simulink model "simulink_flightgear_control_trim_wind_5"  (R2023a)
settings: Solver=VariableStepAuto  StartTime=0  StopTime=inf  FixedStep=0.1  RelTol=1e-3
values from neighbouring files (symbols this model uses):
  alpha = -5:0.1:25    [Boeing747model.m]
  alpha1 = 0:0.1:14    [Boeing747model.m]
  alpha2 = -5:0.1:25    [Boeing747model.m]
  alpha3 = -5:0.1:17    [Boeing747model.m]
  beta = -15:0.1:15    [Boeing747model.m]
  CL = 0:0.01:1.4    [Boeing747model.m]
  da = 0:1:20    [Boeing747model.m]
  dr = [0 5 10 15 20 25]    [Boeing747model.m]
  EPR_ = 0:0.1:1.8    [Boeing747model.m]    (also in engine.m)
  flap = [0 10 20 25 30]    [Boeing747model.m]
  high1 = 0:10000:40000    [Boeing747model.m]
  high2 = 0:20000:40000    [Boeing747model.m]
  high3 = [0 15000 25000 35000 40000]    [Boeing747model.m]    (also in engine.m)
  high4 = [0 10000 20000 40000]    [Boeing747model.m]
  interp_result = table2array(resultTable(:,2:end))    [Boeing747model.m]
  interp_result_mach = 0:0.1:0.9    [Boeing747model.m]
  interp_result_N1 = 80:5:110    [Boeing747model.m]
  m2ft = 3.280839895013    (= 3.28083989501)    [Boeing747model.m]    (also in engine.m)
  mach = 0:0.02:0.9    [Boeing747model.m]    (also in engine.m)
  mach1 = [0 0.3 0.5 0.7 0.8 0.84 0.86 0.88 0.9]    [Boeing747model.m]
  mach2 = [0 0.3 0.5 0.7 0.8 0.9]    [Boeing747model.m]
  mach3 = [0 0.1 0.3 0.5 0.6 0.7 0.8 0.9]    [Boeing747model.m]    (also in engine.m = [0 0.1 0.3 0.5  0.7 0.8 0.9])
  mach5 = [0 0.6 0.8 0.85 0.9]    [Boeing747model.m]
  mach6 = [0 0.6 0.8 0.9]    [Boeing747model.m]
  mach7 = [0 0.3 0.5 0.74 0.8 0.84 0.86 0.88 0.9]    [Boeing747model.m]
  mach8 = [0 0.3 0.5 0.74 0.8 0.84 0.86 0.88 0.9]    [Boeing747model.m]
  model = 'simulink_flightgear_control_trim_wind_5'    [traimcode.m]
  ms2kts = 1.943844492609    (= 1.94384449261)    [Boeing747model.m]    (also in engine.m)
  powerangle_ = 0:1:130    [Boeing747model.m]    (also in engine.m)
  T = [-45 0 60 120]    [Boeing747model.m]    (also in engine.m)
  V_E = 0:20:250    [Boeing747model.m]
undefined symbols (not defined in the file or in its folder): Earth, F, ft, Light, m, MIL, Model, Newton, P3DAERO, Raphson, Receive, s, Send, Unit, WGS84, Wind
libraries: simulink_extras x115, aerolibconvert2 x16, simulink x4, aerolibfltsims x3, shared6dof x1, aerolibasang x1, aerolibtransform2 x1, aerolibatmos2 x1, aerolibobsolete x1, aerolibwind2 x1
(part 5 of 5)

== system simulink_flightgear_control_trim_wind_5/Plane/气动系数/Subsystem58/Subsystem68 ==
  In1 : Inport
  In2 : Inport  Port=2
  Radians in : Inport  Port=3
  In4 : Inport  Port=4
  In5 : Inport  Port=5
  In6 : Inport  Port=6
  1-D Lookup Table54 : Lookup_n-D  NumberOfTableDimensions=1  BreakpointsForDimension1=P3DAERO.Cl_ai_mach(1,:)  Table=P3DAERO.Cl_ai_mach(2,:)  InternalRulePriority=Speed  RndMeth=Simplest
  2-D Lookup Table10 : Lookup_n-D  BreakpointsForDimension1=flap  BreakpointsForDimension2=alpha  Table=P3DAERO.delta_Cl_ai  InternalRulePriority=Speed  RndMeth=Simplest
      settings: InputPortMap=u0,u1
  2-D Lookup Table11 : Lookup_n-D  BreakpointsForDimension1=high1  BreakpointsForDimension2=mach  Table=P3DAERO.Cl_ai_aeroelastic  InternalRulePriority=Speed  RndMeth=Simplest
      settings: InputPortMap=u0,u1
  2-D Lookup Table9 : Lookup_n-D  BreakpointsForDimension1=flap  BreakpointsForDimension2=da  Table=P3DAERO.k_delta_ai  InternalRulePriority=Speed  RndMeth=Simplest
      settings: InputPortMap=u0,u1
  Abs : Abs  SaturateOnIntegerOverflow=off
  Constant16 : Constant  Value=-1
  Constant18 : Constant
  Constant20 : Constant  Value=2
  Gain3 : Gain  Gain=m2ft
  Product4 : Product  Inputs=3
  Product5 : Product  Inputs=5
  Radians to Degrees26 : simulink_extras/Transformations/Radians to Degrees
  Radians to Degrees9 : simulink_extras/Transformations/Radians to Degrees
  Saturation8 : Saturate  UpperLimit=20  LowerLimit=0
  Scope1 : Scope
  Scope4 : Scope
  Switch2 : Switch  SaturateOnIntegerOverflow=off  InputSameDT=off
  Out1 : Outport
  wires:
  In5/1 -> Switch2/2, Abs/1
  1-D Lookup Table54/1 -> Product5/1
  Switch2/1 -> Product4/3
  2-D Lookup Table10/1 -> Product5/2
  2-D Lookup Table11/1 -> Product5/3
  2-D Lookup Table9/1 -> Product5/4
  Radians to Degrees26/1 -> Saturation8/1
  In1/1 -> 2-D Lookup Table11/2, 1-D Lookup Table54/1
  In6/1 -> Product5/5
  Gain3/1 -> 2-D Lookup Table11/1
  Product5/1 -> Scope4/1, Product4/2
  Radians to Degrees9/1 -> 2-D Lookup Table10/2
  Constant16/1 -> Switch2/1
  In2/1 -> 2-D Lookup Table9/1, 2-D Lookup Table10/1
  Saturation8/1 -> 2-D Lookup Table9/2
  Constant20/1 -> Product4/1
  Constant18/1 -> Switch2/3
  Radians in/1 -> Radians to Degrees9/1
  In4/1 -> Gain3/1
  Product4/1 -> Scope1/1, Out1/1
  Abs/1 -> Radians to Degrees26/1

== system simulink_flightgear_control_trim_wind_5/Plane/气动系数/Subsystem58/Subsystem69 ==
  In1 : Inport
  Radians in : Inport  Port=2
  Gain : Gain  Gain=-0.0003
  Product15 : Product
  Radians to Degrees2 : simulink_extras/Transformations/Radians to Degrees
  Scope47 : Scope
  Out1 : Outport
  wires:
  Gain/1 -> Product15/2
  Radians to Degrees2/1 -> Gain/1
  Product15/1 -> Out1/1, Scope47/1
  Radians in/1 -> Radians to Degrees2/1
  In1/1 -> Product15/1

== system simulink_flightgear_control_trim_wind_5/Plane/气动系数/Subsystem58/Subsystem7 ==
  note: 低速模式
  note: 高速模式
  In1 : Inport
  In2 : Inport  Port=2
  In3 : Inport  Port=3
  In4 : Inport  Port=4
  In5 : Inport  Port=5
  2-D Lookup Table6 : Lookup_n-D  BreakpointsForDimension1=flap  BreakpointsForDimension2=V_E  Table=P3DAERO.dot_CL_dot_nz_lowspeed  InternalRulePriority=Speed  RndMeth=Simplest
      settings: InputPortMap=u0,u1
  2-D Lookup Table7 : Lookup_n-D  BreakpointsForDimension1=high1  BreakpointsForDimension2=mach  Table=P3DAERO.dot_CL_dot_nz_highspeed  InternalRulePriority=Speed  RndMeth=Simplest
      settings: InputPortMap=u0,u1
  Product4 : Product
  Scope7 : Scope
  Velocity Conversion : aerolibconvert2/Velocity Conversion  IU=m/s  OU=ft/s
  Out1 : Outport
  wires:
  In5/1 -> 2-D Lookup Table7/2
  Product4/1 -> Out1/1, Scope7/1
  In2/1 -> 2-D Lookup Table6/1
  In3/1 -> 2-D Lookup Table6/2
  2-D Lookup Table7/1 -> Product4/2
  In1/1 -> Product4/1
  In4/1 -> Velocity Conversion/1
  Velocity Conversion/1 -> 2-D Lookup Table7/1

== system simulink_flightgear_control_trim_wind_5/Plane/气动系数/Subsystem58/Subsystem8 ==
  note: 米变英尺
  note: 襟翼角度
  In1 : Inport
  In2 : Inport  Port=2
  Radians in : Inport  Port=3
  1-D Lookup Table97 : Lookup_n-D  NumberOfTableDimensions=1  BreakpointsForDimension1=P3DAERO.k_ge(1,:)  Table=P3DAERO.k_ge(2,:)  InternalRulePriority=Speed  RndMeth=Simplest
  2-D Lookup Table18 : Lookup_n-D  BreakpointsForDimension1=flap  BreakpointsForDimension2=alpha1  Table=P3DAERO.delta_CL_ge  InternalRulePriority=Speed  RndMeth=Simplest
      settings: InputPortMap=u0,u1
  Constant24 : Constant  Value=0
  Product16 : Product
  Radians to Degrees10 : simulink_extras/Transformations/Radians to Degrees
  Saturation3 : Saturate  UpperLimit=14  LowerLimit=0
  Scope48 : Scope
  Scope49 : Scope
  Switch12 : Switch  Criteria=u2 > Threshold  Threshold=24  SaturateOnIntegerOverflow=off  InputSameDT=off
  Velocity Conversion : aerolibconvert2/Velocity Conversion  IU=m/s  OU=ft/s
  Out1 : Outport
  wires:
  Radians to Degrees10/1 -> Saturation3/1
  Product16/1 -> Switch12/3
  Velocity Conversion/1 -> 1-D Lookup Table97/1
  Constant24/1 -> Switch12/1
  Saturation3/1 -> 2-D Lookup Table18/2
  Switch12/1 -> Out1/1, Scope49/1
  2-D Lookup Table18/1 -> Product16/2
  1-D Lookup Table97/1 -> Product16/1, Scope48/1
  Radians in/1 -> Radians to Degrees10/1
  In2/1 -> 2-D Lookup Table18/1
  In1/1 -> Velocity Conversion/1, Switch12/2

== system simulink_flightgear_control_trim_wind_5/Plane/气动系数/Subsystem58/Subsystem9 ==
  note: 地效修正
  note: 米变英尺
  note: 襟翼角度
  In1 : Inport
  In2 : Inport  Port=2
  Radians in : Inport  Port=3
  1-D Lookup Table59 : Lookup_n-D  NumberOfTableDimensions=1  BreakpointsForDimension1=P3DAERO.k_ge(1,:)  Table=P3DAERO.k_ge(2,:)  InternalRulePriority=Speed  RndMeth=Simplest
  2-D Lookup Table12 : Lookup_n-D  BreakpointsForDimension1=flap  BreakpointsForDimension2=alpha1  Table=P3DAERO.F_rho_ge  InternalRulePriority=Speed  RndMeth=Simplest
      settings: InputPortMap=u0,u1
  Constant18 : Constant
  Product12 : Product
  Radians to Degrees6 : simulink_extras/Transformations/Radians to Degrees
  Saturation1 : Saturate  UpperLimit=14  LowerLimit=0
  Scope31 : Scope
  Scope33 : Scope
  Sum11 : Sum
  Switch4 : Switch  Criteria=u2 > Threshold  Threshold=24  SaturateOnIntegerOverflow=off  InputSameDT=off
  Velocity Conversion : aerolibconvert2/Velocity Conversion  IU=m/s  OU=ft/s
  Out1 : Outport
  Out2 : Outport  Port=2
  wires:
  In2/1 -> 2-D Lookup Table12/1
  Radians to Degrees6/1 -> Saturation1/1
  Switch4/1 -> Out1/1, Scope31/1
  Velocity Conversion/1 -> 1-D Lookup Table59/1
  Saturation1/1 -> 2-D Lookup Table12/2
  Sum11/1 -> Switch4/3
  Constant18/1 -> Sum11/1, Switch4/1
  2-D Lookup Table12/1 -> Product12/1
  1-D Lookup Table59/1 -> Product12/2, Out2/1, Scope33/1
  Product12/1 -> Sum11/2
  Radians in/1 -> Radians to Degrees6/1
  In1/1 -> Velocity Conversion/1, Switch4/2

== matlab function simulink_flightgear_control_trim_wind_5/Plane/发动机/MATLAB Function2 ==
  data: flap input; site output; ma input
function site= fcn(flap,ma)
if(ma>=0&&ma<=0.25)
    if(flap==0)
    site=0;
    elseif (flap>0.1&&flap<=0.25)
        site=1;
    elseif(flap>0.25&&flap<=0.5)
        site=2;
    elseif(flap>0.5&&flap<=0.75)
        site=3;
    elseif(flap>0.75&&flap<=1)
        site=4;
    else
    site=0;
    end
elseif(ma>0.25&&ma<=0.35)
    if(flap==0)
    site=0;
    elseif(flap>0.1&&flap<=0.25)
        site=1;
    elseif(flap>0.25&&flap<=0.5)
        site=2;
    elseif(flap>0.5)
        site=3;
    else
    site=0;
    end
else
    site=0;
end

== matlab function simulink_flightgear_control_trim_wind_5/Plane/重量//惯量/MATLAB Function1 ==
  data: ixx input; y output; iyy input; izz input; ixz input
function y = fcn(ixx,iyy,izz,ixz)
I=[ixx  0  -ixz;
    0  iyy  0;
    -ixz 0   izz];
y = I;

== matlab function simulink_flightgear_control_trim_wind_5/Plane/MATLAB Function ==
  data: u input; y output
function y = fcn(u)

y = [(25-u)/100*8.32,0,0]';

== matlab function simulink_flightgear_control_trim_wind_5/Plane/气动系数/MATLAB Function ==
  data: u input; y output
function y = fcn(u)

x = [cosd(u) 0 -sind(u); %x为稳定轴系到体轴系的转换
    0       1      0 ;
    sind(u) 0  cosd(u)];

y=x';                  %y为体轴系到稳定轴系的转换

== matlab function simulink_flightgear_control_trim_wind_5/Plane/大气环境/气压高度+摄氏度偏差版本1 ==
  data: T output; p output; rho output; Hp input; a output; delta_ISA input; delta output; theta output; sigma output; Hd_m output; Hd_ft output
% File: isa_atmosphere_pressure_altitude_delta.m
%
% 输入:
%   Hp        气压高度 / pressure altitude (m) [0–84.852 km]
%   delta_ISA 温度偏差 (degC)，比如 -40 表示 ISA -40
%
% 输出:
%   T     实际温度 (K)，即 T_ISA(Hp) + delta_ISA
%   p     静压 (Pa)，由气压高度按 ISA 标准大气确定
%   rho   实际密度 (kg/m^3)，由 p 和 T 计算
%   a     实际声速 (m/s)，由 T 计算
%   delta 压力比 p/p0
%   theta 温度比 T/T0
%   sigma 密度比 rho/rho0
%   Hd_m  密度高度 (m)
%   Hd_ft 密度高度 (ft)

function [T, p, rho, a, delta, theta, sigma, Hd_m, Hd_ft] = isa_atmosphere_pressure_altitude_delta(Hp, delta_ISA)

    % 常数
    g0 = 9.80665;        % m/s^2
    R  = 287.05287;      % J/(kg*K)
    gamma = 1.4;         % 空气比热比

    p0 = 101325;         % Pa
    T0 = 288.15;         % K
    rho0 = 1.225;        % kg/m^3

    % ISA 分层参数
    h_base = [0, 11000, 20000, 32000, 47000, 51000, 71000, 84852]; % m
    L      = [-0.0065, 0.0, 0.0010, 0.0028, 0.0, -0.0028, -0.0020]; % K/m

    % 输入检查
    if any(Hp(:) < 0) || any(Hp(:) > 84852)
        error('Hp must be within [0, 84852] m.');
    end

    if isscalar(delta_ISA)
        delta_ISA = delta_ISA .* ones(size(Hp));
    elseif ~isequal(size(delta_ISA), size(Hp))
        error('delta_ISA must be scalar or the same size as Hp.');
    end

    T_ISA = zeros(size(Hp));
    p     = zeros(size(Hp));

    % 对每一个气压高度计算 ISA 温度和 ISA 压力
    for i = 1:numel(Hp)

        h = Hp(i);

        T_curr = T0;
        p_curr = p0;

        for j = 1:length(L)

            h1 = h_base(j);
            h2 = h_base(j+1);

            if h <= h2

                if L(j) == 0
                    T_layer = T_curr;
                    p(i) = p_curr * exp(-g0 * (h - h1) / (R * T_layer));
                else
                    T_layer = T_curr + L(j) * (h - h1);
                    p(i) = p_curr * (T_layer / T_curr)^(-g0 / (R * L(j)));
                end

                T_ISA(i) = T_layer;
                break;

            else

                if L(j) == 0
                    T_next = T_curr;
                    p_curr = p_curr * exp(-g0 * (h2 - h1) / (R * T_curr));
                else
                    T_next = T_curr + L(j) * (h2 - h1);
                    p_curr = p_curr * (T_next / T_curr)^(-g0 / (R * L(j)));
                end

                T_curr = T_next;
            end
        end
    end

    % 实际温度：ISA 温度 + ΔISA
    T = T_ISA + delta_ISA;

    if any(T(:) <= 0)
        error('Computed temperature is non-physical. T must be greater than 0 K.');
    end

    % 实际密度和声速
    rho = p ./ (R .* T);
    a   = sqrt(gamma * R .* T);

    % 无量纲比值
    delta = p ./ p0;
    theta = T ./ T0;
    sigma = rho ./ rho0;

    % 密度高度
    Hd_m = density_altitude_from_rho(rho);
    Hd_ft = Hd_m * 3.280839895;
end


function Hd = density_altitude_from_rho(rho_target)

    h_low  = -3048;   % -10000 ft
    h_high = 15240;   %  50000 ft

    Hd = zeros(size(rho_target));

    for i = 1:numel(rho_target)
        lo = h_low;
        hi = h_high;

        for k = 1:60
            mid = 0.5 * (lo + hi);
            rho_mid = isa_density(mid);

            if rho_mid > rho_target(i)
                lo = mid;
            else
                hi = mid;
            end
        end

        Hd(i) = 0.5 * (lo + hi);
    end
end


function rho = isa_density(h)
    [T, p] = isa_standard_Tp(h);
    R = 287.05287;
    rho = p / (R * T);
end


function [T, p] = isa_standard_Tp(h)

    g0 = 9.80665;
    R  = 287.05287;

    p0 = 101325;
    T0 = 288.15;

    h_base = [0, 11000, 20000, 32000, 47000, 51000, 71000, 84852];
    L      = [-0.0065, 0.0, 0.0010, 0.0028, 0.0, -0.0028, -0.0020];

    % 默认赋值，避免 Simulink Coder 认为输出未赋值
    T = T0;
    p = p0;

    T_curr = T0;
    p_curr = p0;

    for j = 1:length(L)
        h1 = h_base(j);
        h2 = h_base(j+1);

        if h <= h2
            if L(j) == 0
                T = T_curr;
                p = p_curr * exp(-g0 * (h - h1) / (R * T));
            else
                T = T_curr + L(j) * (h - h1);
                p = p_curr * (T / T_curr)^(-g0 / (R * L(j)));
            end
            return;
        else
            if L(j) == 0
                T_next = T_curr;
                p_curr = p_curr * exp(-g0 * (h2 - h1) / (R * T_curr));
            else
                T_next = T_curr + L(j) * (h2 - h1);
                p_curr = p_curr * (T_next / T_curr)^(-g0 / (R * L(j)));
            end

            T_curr = T_next;
        end
    end

    % 兜底路径，给 Coder 明确输出
    T = T_curr;
    p = p_curr;
end

== matlab function simulink_flightgear_control_trim_wind_5/Plane/气动系数/Subsystem58/Subsystem32/MATLAB Function15 ==
  data: u input; y output
function y = fcn(u)
%计算kq
y=-0.012*(u-25)+1;

== matlab function simulink_flightgear_control_trim_wind_5/Plane/大气环境/气压高度+摄氏度偏差版本 ==
  data: T output; p output; rho output; Hp input; a output; delta_ISA input; delta output; theta output; sigma output
% File: isa_atmosphere_pressure_altitude_delta.m
%
% 输入:
%   Hp        气压高度 / pressure altitude (m) [0–84.852 km]
%   delta_ISA 温度偏差 (°C)，比如 -40 表示 ISA -40
%
% 输出:
%   T     实际温度 (K)，即 T_ISA(Hp) + delta_ISA
%   p     静压 (Pa)，由气压高度按 ISA 标准大气确定
%   rho   实际密度 (kg/m^3)，由 p 和 T 计算
%   a     实际声速 (m/s)，由 T 计算
%
% 可选输出:
%   delta 压力比 p/p0
%   theta 温度比 T/T0
%   sigma 密度比 rho/rho0

function [T, p, rho, a, delta, theta, sigma] = isa_atmosphere_pressure_altitude_delta(Hp, delta_ISA)

    % 常数
    g0 = 9.80665;        % m/s^2
    R  = 287.05287;      % J/(kg·K)
    gamma = 1.4;         % 空气比热比

    p0 = 101325;         % Pa
    T0 = 288.15;         % K
    rho0 = 1.225;        % kg/m^3

    % ISA 分层参数
    % 注意：这里 Hp 按标准大气的高度层处理
    h_base = [0, 11000, 20000, 32000, 47000, 51000, 71000, 84852]; % m
    L      = [-0.0065, 0.0, 0.0010, 0.0028, 0.0, -0.0028, -0.0020]; % K/m

    % 输入检查
    if any(Hp(:) < 0) || any(Hp(:) > 84852)
        error('Hp must be within [0, 84852] m.');
    end

    % 允许 delta_ISA 为标量或与 Hp 同尺寸
    if isscalar(delta_ISA)
        delta_ISA = delta_ISA .* ones(size(Hp));
    elseif ~isequal(size(delta_ISA), size(Hp))
        error('delta_ISA must be scalar or the same size as Hp.');
    end

    % 初始化
    T_ISA = zeros(size(Hp));
    p     = zeros(size(Hp));

    % 对每一个气压高度计算 ISA 温度和 ISA 压力
    for i = 1:numel(Hp)

        h = Hp(i);

        % 这里不能加 delta_ISA
        % 因为 pressure altitude 对应的压力必须由标准 ISA 反算
        T_curr = T0;
        p_curr = p0;

        for j = 1:length(L)

            h1 = h_base(j);
            h2 = h_base(j+1);

            if h <= h2

                if L(j) == 0
                    % 等温层
                    T_layer = T_curr;
                    p(i) = p_curr * exp(-g0 * (h - h1) / (R * T_layer));
                else
                    % 温度梯度层
                    T_layer = T_curr + L(j) * (h - h1);
                    p(i) = p_curr * (T_layer / T_curr)^(-g0 / (R * L(j)));
                end

                T_ISA(i) = T_layer;
                break;

            else

                % 穿越完整一层，更新到下一层基准
                if L(j) == 0
                    T_next = T_curr;
                    p_curr = p_curr * exp(-g0 * (h2 - h1) / (R * T_curr));
                else
                    T_next = T_curr + L(j) * (h2 - h1);
                    p_curr = p_curr * (T_next / T_curr)^(-g0 / (R * L(j)));
                end

                T_curr = T_next;
            end
        end
    end

    % 实际温度：在气压高度对应的 ISA 温度基础上加 ΔISA
    T = T_ISA + delta_ISA;

    if any(T(:) <= 0)
        error('Computed temperature is non-physical. T must be greater than 0 K.');
    end

    % 用实际温度计算密度和声速
    rho = p ./ (R .* T);
    a   = sqrt(gamma * R .* T);

    % 常用无量纲比值
    delta = p ./ p0;       % 压力比
    theta = T ./ T0;       % 温度比
    sigma = rho ./ rho0;   % 密度比
end

== matlab function simulink_flightgear_control_trim_wind_5/Plane/气动系数/Subsystem58/Subsystem44/MATLAB Function3 ==
  data: u input; y output
function y = fcn(u)
y=-0.004*(u-25);

== matlab function simulink_flightgear_control_trim_wind_5/Plane/气动系数/Subsystem58/Subsystem44/MATLAB Function2 ==
  data: u input; y output
function y = fcn(u)
y=-0.004*(u-25)+1;

== matlab function simulink_flightgear_control_trim_wind_5/Plane/气动力//力矩/MATLAB Function ==
  data: u input; y output
function y = fcn(u)

x = [cosd(u) 0 -sind(u); %x为稳定轴系到体轴系的转换
    0       1      0 ;
    sind(u) 0  cosd(u)];

y=x;

== matlab function simulink_flightgear_control_trim_wind_5/Plane/发动机/MATLAB Function4 ==
  data: u input; y output
function y = fcn(u)

y = u*9/5-459.67;

== matlab function simulink_flightgear_control_trim_wind_5/Plane/气动系数/Subsystem58/Subsystem6/MATLAB Function15 ==
  data: u input; y output
function y = fcn(u)
%计算kq
y = -0.018*u+1.45;

== matlab function simulink_flightgear_control_trim_wind_5/Plane/发动机/MATLAB Function ==
  data: x input; T output; y input; z input
function T = fcn(x,y,z)

T= [x,y,z]';

== matlab function simulink_flightgear_control_trim_wind_5/Plane/发动机/MATLAB Function1 ==
  data: x input; MT output; y input; z input
function MT = fcn(x,y,z)

MT= [x,y,z]';
